simulink model "vehicle_base"  (R2026b)
settings: Solver=ode3  StopTime=tEnd  FixedStep=0.1
undefined symbols (not defined in the file): Fmax, g, Ki, Kp, rho, veh_A, veh_Cd, veh_Crr, veh_m
settings Model: Creator=Hamza  LastModifiedBy=Hamza

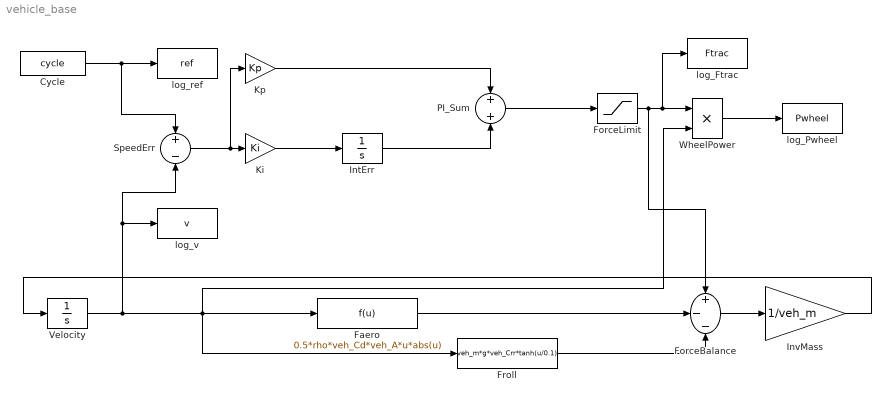
== system vehicle_base ==
  Cycle : FromWorkspace  VariableName=cycle
  Faero : Fcn  Expr=0.5*rho*veh_Cd*veh_A*u*abs(u)
  ForceBalance : Sum  Inputs=+--
  ForceLimit : Saturate  UpperLimit=Fmax  LowerLimit=-Fmax
  Froll : Fcn  Expr=veh_m*g*veh_Crr*tanh(u/0.1)
  IntErr : Integrator  LimitOutput=on  UpperSaturationLimit=Fmax  LowerSaturationLimit=-Fmax
  InvMass : Gain  Gain=1/veh_m
  Ki : Gain  Gain=Ki
  Kp : Gain  Gain=Kp
  PI_Sum : Sum
  SpeedErr : Sum  Inputs=+-
  Velocity : Integrator
  WheelPower : Product
  log_Ftrac : ToWorkspace  VariableName=Ftrac  SaveFormat=Timeseries  SampleTime=-1
  log_Pwheel : ToWorkspace  VariableName=Pwheel  SaveFormat=Timeseries  SampleTime=-1
  log_ref : ToWorkspace  VariableName=ref  SaveFormat=Timeseries  SampleTime=-1
  log_v : ToWorkspace  VariableName=v  SaveFormat=Timeseries  SampleTime=-1
  wires:
  Faero/1 -> ForceBalance/2
  Velocity/1 -> Froll/1, Faero/1, WheelPower/2, SpeedErr/2, log_v/1
  Cycle/1 -> SpeedErr/1, log_ref/1
  Ki/1 -> IntErr/1
  Kp/1 -> PI_Sum/1
  SpeedErr/1 -> Kp/1, Ki/1
  IntErr/1 -> PI_Sum/2
  PI_Sum/1 -> ForceLimit/1
  InvMass/1 -> Velocity/1
  ForceBalance/1 -> InvMass/1
  Froll/1 -> ForceBalance/3
  ForceLimit/1 -> WheelPower/1, log_Ftrac/1, ForceBalance/1
  WheelPower/1 -> log_Pwheel/1
